simulink model "Exp2"  (R2025b)
settings: Solver=VariableStepAuto  StartTime=0.0  StopTime=10.0  RelTol=1e-3
settings Model: Creator=SUBHASH  LastModifiedBy=SUBHASH

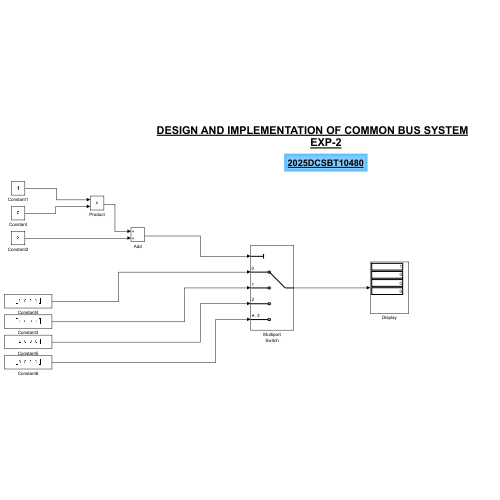
[thumbnail: Simulink's stored preview of the top-level diagram]
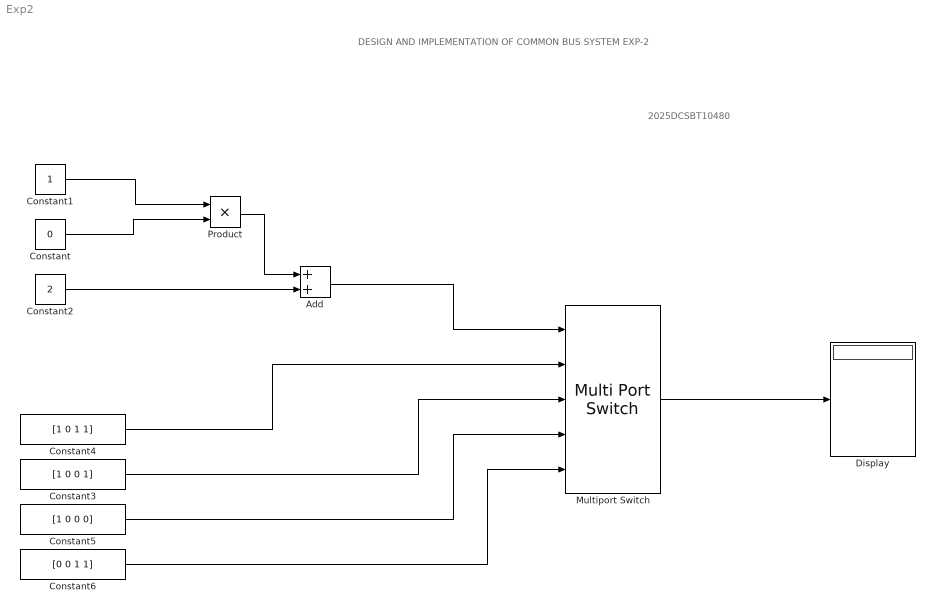
== system Exp2 ==
  note: 2025DCSBT10480
  note: DESIGN AND IMPLEMENTATION OF COMMON BUS SYSTEM
      | EXP-2
  Add : Sum
  Constant : Constant  Value=0
  Constant1 : Constant
  Constant2 : Constant  Value=2
  Constant3 : Constant  Value=[1 0 0 1]
  Constant4 : Constant  Value=[1 0 1 1]
  Constant5 : Constant  Value=[1 0 0 0]
  Constant6 : Constant  Value=[0 0 1 1]
  Display : Display
  Multiport Switch : MultiPortSwitch  DataPortOrder=Zero-based contiguous  Inputs=4  zeroidx=on  SaturateOnIntegerOverflow=off  InputSameDT=off
  Product : Product
  wires:
  Constant1/1 -> Product/1
  Constant/1 -> Product/2
  Constant2/1 -> Add/2
  Product/1 -> Add/1
  Add/1 -> Multiport Switch/1
  Constant4/1 -> Multiport Switch/2
  Constant3/1 -> Multiport Switch/3
  Constant5/1 -> Multiport Switch/4
  Constant6/1 -> Multiport Switch/5
  Multiport Switch/1 -> Display/1
